simulink model "SpeedReference"  (R2026b)
settings: Solver=VariableStepAuto
values from neighbouring files (symbols this model uses):
  Ref_Min = -1500    [DCMotorParams.m]
  Ref_Period = 2    [DCMotorParams.m]
  Ref_Start = 1500    [DCMotorParams.m]
  Ref_Step = 150    [DCMotorParams.m]
  Ts = 0.01    [DCMotorParams.m]
settings Model: Creator=bence  LastModifiedBy=bence

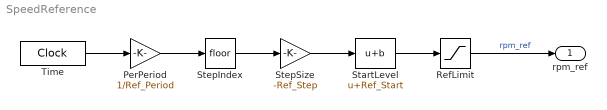
== system SpeedReference ==
  PerPeriod : Gain  Gain=1/Ref_Period
  RefLimit : Saturate  UpperLimit=Ref_Start  LowerLimit=Ref_Min
  StartLevel : Bias  Bias=Ref_Start  SaturateOnIntegerOverflow=off
  StepIndex : Rounding
  StepSize : Gain  Gain=-Ref_Step
  Time : DigitalClock  SampleTime=Ts
  rpm_ref : Outport
  wires:
  RefLimit/1 -> rpm_ref/1  "rpm_ref"
  StartLevel/1 -> RefLimit/1
  StepSize/1 -> StartLevel/1
  StepIndex/1 -> StepSize/1
  PerPeriod/1 -> StepIndex/1
  Time/1 -> PerPeriod/1
